simulink model "tb_power_plant"  (R2026b)
model workspace (MAT data in the model file):
  TB.do0_t = [0 0.01 10000000]
  TB.do0_v = [0 1 1]
  TB.do1_t = [0 0.03 0.08 10000000]
  TB.do1_v = [0 1 0 0]
  TB.k3_t = [0 10000000]
  TB.k3_v = [0 0]
  TB.duty_t = [0 10000000]
  TB.duty_v = [0 0]
  TB.noz_t = [0 10000000]
  TB.noz_v = [0 0]
  TB.lift_t = [0 10000000]
  TB.lift_v = [0 0]
  TB.estopF_t = [0 10000000]
  TB.estopF_v = [0 0]
  TB.estopR_t = [0 10000000]
  TB.estopR_v = [0 0]
  TB.wless_t = [0 10000000]
  TB.wless_v = [0 0]
  TB.bumpF_t = [0 10000000]
  TB.bumpF_v = [0 0]
  TB.bumpR_t = [0 10000000]
  TB.bumpR_v = [0 0]
  TB.reset_t = [0 10000000]
  TB.reset_v = [0 0]
  TB.keyoff_t = [0 10000000]
  TB.keyoff_v = [0 0]
  TB.ch2_t = [0 10000000]
  TB.ch2_v = [0 0]
  TB.bmsf_t = [0 10000000]
  TB.bmsf_v = [0 0]
  TB.hv_t = [0 1 10000000]
  TB.hv_v = [0 1 1]
  TB.chg_t = [0 10000000]
  TB.chg_v = [0 0]
  TB.rst_t = [0 10000000]
  TB.rst_v = [0 0]
  TB.sd_t = [0 10000000]
  TB.sd_v = [0 0]
  TB.alive_freeze_t = 1000000000
  TB.ien_t = [0 10000000]
  TB.ien_v = [0 0]
  TB.ispd_t = [0 10000000]
  TB.ispd_v = [0 0]
  TB.icmd_stop_t = 1000000000
  TB.P24_t = [0 10000000]
  TB.P24_v = [53 53]
  TB.P12_t = [0 10000000]
  TB.P12_v = [99 99]
  TB.P5_t = [0 10000000]
  TB.P5_v = [2.5 2.5]
  TB.P3_t = [0 10000000]
  TB.P3_v = [0.6 0.6]
  TB.T_amb = 298.15
  TB.G_solar = 0
  TB.dock_t = [0 10000000]
  TB.dock_v = [0 0]
  TB.C_drv = 0.0022
  TB.R_esr = 0.01
  TB.loadL_t = [0 10000000]
  TB.loadL_v = [0 0]
  TB.loadR_t = [0 10000000]
  TB.loadR_v = [0 0]
  TB.load_is_power = 0
  TB.V_gate = [30 35]
  TB.short_t = [0 10000000]
  TB.short_v = [0 0]
  TB.R_short = 0.005
  TB.J_impl = 0.05
  TB.k_aero = 1.19e-05
  TB.k_lin = 0
  TB.T_c = 0
  TB.k_lf = 0
  TB.lf_t = [0 10000000]
  TB.lf_v = [1 1]
  TB.p_line = 0
  TB.MaxNonlinIter = 3
  TB.MaxModeIter = 2
  TB.dec_fast = 1
  TB.dec_slow = 1
  TB.dec_bms = 1
  TB.dec_truth = 1
values from neighbouring files (symbols this model uses):
  P = local_temp(P, 318.15)    [pwr_case_def.m]    (also in pwr_case_run.m = C.pmod(P))
undefined symbols (not defined in the file or in its folder): bms_fault, estop_ch2_stuck, linePressure, shaftSpeed, shaftTorque, Ts, type, VC_IMPL
libraries: simulink x21, fl_lib x9, nesl_utility x8, ee_lib x4
settings Model: Creator=aomar  LastModifiedBy=aomar

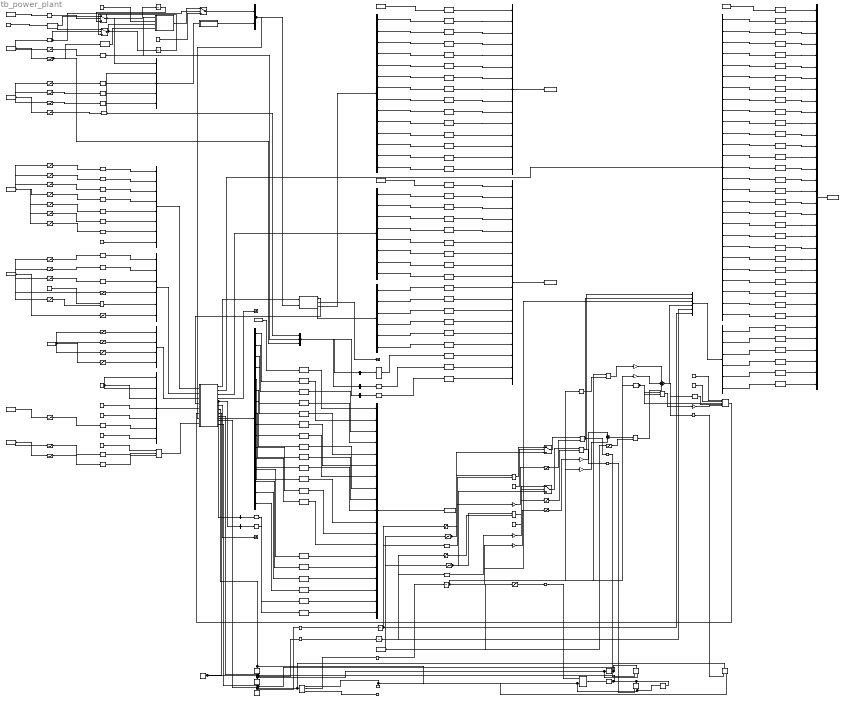
== system tb_power_plant ==
  Alive_cnt : simulink/Sources/Counter Free-Running  NumBits=8  tsamp=Ts.can_slow
  Alive_u8 : DataTypeConversion  OutDataTypeStr=uint8  SaturateOnIntegerOverflow=off  RndMeth=Floor
  Angle_term : fl_lib/Physical Signals/Sinks/PS Terminator
  BMS : ModelReference  ModelNameDialog=Shaddad_BMS  SimulationMode=Normal  ModelReferenceVersion=1.1
  BMS_REQ_Pack : Subsystem  ReferencedSubsystem=bmsreq_can_pack
  BmsReq_BC : BusCreator  Inputs=5  OutDataTypeStr=Bus: Bus_BmsReq  NonVirtualBus=on
      settings: InheritFromInputs=off
  Bms_alive_hold : UnitDelay  InitialCondition=uint8(0)  SampleTime=Ts.can_slow
  Bms_alive_run : simulink/Logic and Bit Operations/Compare To Constant  relop=<  const=TB.alive_freeze_t  OutDataTypeStr=boolean
  Bms_alive_sw : Switch  Criteria=u2 ~= 0  SaturateOnIntegerOverflow=off  InputSameDT=off
  C_drv_L : ee_lib/Passive/Capacitor  cap_option=ee.enum.passive.capacitor.capOption.const  c=TB.C_drv F  Cvec=[1e-05, 1e-06] F  Vvec=[0, 10] V  CV_table_symmetry=ee.enum.passive.capacitor.tableSymmetry.yes  f_vec=[1, 10] kHz  DFext_vec=[.8, 1.2]  enable_C_tol=ee.enum.toleranceApplication.none  averaging_period=0 s  C_tol=5  tol_distribution=ee.enum.toleranceDistribution.uniform  nSigma=4  r=TB.R_esr Ohm  g=0 1/Ohm  enable_operating_limits=ee.enum.enable.no  operating_limit_action=ee.enum.passive.reportOpLim.warn  max_working_voltage_range=[-25, 25] V  power_rating=1 W  maxTemperature=85 degC  thermalEnable=false  thermalMass=1 J/K  i_specify=off  i_priority=None  i=0 A  i_nominal_specify=off  i_nominal_value=1  i_nominal_unit=A  v_specify=off  v_priority=None  v=0 V  v_nominal_specify=off  v_nominal_value=1  v_nominal_unit=V  vc_specify=on  vc_priority=High  vc=0 V  vc_nominal_specify=off  vc_nominal_value=1  vc_nominal_unit=V  T_specify=off  T_priority=None  T=298.15 K  T_nominal_specify=off  T_nominal_value=1  T_nominal_unit=K
  C_drv_R : ee_lib/Passive/Capacitor  cap_option=ee.enum.passive.capacitor.capOption.const  c=TB.C_drv F  Cvec=[1e-05, 1e-06] F  Vvec=[0, 10] V  CV_table_symmetry=ee.enum.passive.capacitor.tableSymmetry.yes  f_vec=[1, 10] kHz  DFext_vec=[.8, 1.2]  enable_C_tol=ee.enum.toleranceApplication.none  averaging_period=0 s  C_tol=5  tol_distribution=ee.enum.toleranceDistribution.uniform  nSigma=4  r=TB.R_esr Ohm  g=0 1/Ohm  enable_operating_limits=ee.enum.enable.no  operating_limit_action=ee.enum.passive.reportOpLim.warn  max_working_voltage_range=[-25, 25] V  power_rating=1 W  maxTemperature=85 degC  thermalEnable=false  thermalMass=1 J/K  i_specify=off  i_priority=None  i=0 A  i_nominal_specify=off  i_nominal_value=1  i_nominal_unit=A  v_specify=off  v_priority=None  v=0 V  v_nominal_specify=off  v_nominal_value=1  v_nominal_unit=V  vc_specify=on  vc_priority=High  vc=0 V  vc_nominal_specify=off  vc_nominal_value=1  vc_nominal_unit=V  T_specify=off  T_priority=None  T=298.15 K  T_nominal_specify=off  T_nominal_value=1  T_nominal_unit=K
  CanSlow_BC : BusCreator  Inputs=2  OutDataTypeStr=Bus: Bus_Can1_McuSlow  NonVirtualBus=on
      settings: InheritFromInputs=off
  Clock_100ms : DigitalClock  SampleTime=Ts.env
  Clock_100ms_log : DigitalClock  SampleTime=Ts.hk
  Clock_100ms_log_bms : DigitalClock  SampleTime=Ts.hk
  Clock_10ms : DigitalClock  SampleTime=Ts.ctrl
  Clock_10ms_lv : DigitalClock  SampleTime=Ts.ctrl
  Clock_50ms : DigitalClock  SampleTime=Ts.can_slow
  Clock_50ms_alive : DigitalClock  SampleTime=Ts.can_slow
  Clock_50ms_impl : DigitalClock  SampleTime=Ts.can_slow
  Clock_base : DigitalClock  SampleTime=Ts.base
  Clock_base_flt : DigitalClock  SampleTime=Ts.base
  Clock_base_hmi : DigitalClock  SampleTime=Ts.base
  Clock_base_hw : DigitalClock  SampleTime=Ts.base
  Clock_base_stub : DigitalClock  SampleTime=Ts.base
  Cmd_sel : BusSelector  OutputSignals=K1_Cmd,K2_Cmd,K4_Cmd,Charger_Enable,Charger_I_Req_A,Fan_Cmd
  Dist : Constant  Value=0  SampleTime=Ts.env
  Env_BC : BusCreator  Inputs=7  OutDataTypeStr=Bus: Bus_EnvState  NonVirtualBus=on
      settings: InheritFromInputs=off
  Flt_BA : BusAssignment  AssignedSignals=estop_ch2_stuck,bms_fault
  Flt_ic : Constant  Value=P.ic.Bus_FaultInject  OutDataTypeStr=Bus: Bus_FaultInject  SampleTime=Ts.base
  G_solar : Constant  Value=TB.G_solar  SampleTime=Ts.env
  Gate_L : Saturate  UpperLimit=1  LowerLimit=0
  Gate_L_k : Gain  Gain=1/(TB.V_gate(2) - TB.V_gate(1))
  Gate_L_off : Bias  Bias=-TB.V_gate(1)  SaturateOnIntegerOverflow=off
  Gate_R : Saturate  UpperLimit=1  LowerLimit=0
  Gate_R_k : Gain  Gain=1/(TB.V_gate(2) - TB.V_gate(1))
  Gate_R_off : Bias  Bias=-TB.V_gate(1)  SaturateOnIntegerOverflow=off
  Hmi_BC : BusCreator  Inputs=8  OutDataTypeStr=Bus: Bus_HmiInputs  NonVirtualBus=on
      settings: InheritFromInputs=off
  Hv_RT : RateTransition  OutPortSampleTime=Ts.ctrl
  Hv_log_sel : BusSelector  OutputSignals=HV_Enable_Req
  Hw_BC : BusCreator  Inputs=6  OutDataTypeStr=Bus: Bus_PowerHwCmd  NonVirtualBus=on
      settings: InheritFromInputs=off
  IMPL_CMD_Pack : Subsystem  ReferencedSubsystem=implcmd_can_pack
  I_drv_L : fl_lib/Electrical/Electrical Sources/Controlled Current Source
  I_drv_L_PS : nesl_utility/Simulink-PS Converter  PhysicalDomain=network_engine_domain  SubClassName=ps_input  LeftPortType=input  RightPortType=output  PseudoPeriodic=off  Frequencies=[]  NoiseDistribution=none  NoiseParameters=[]  Unit=A  AffineConversion=off  FilteringAndDerivatives=zero  SimscapeFilterOrder=1  InputFilterTimeConstant=0.001  UdotUserProvided=0
  I_drv_R : fl_lib/Electrical/Electrical Sources/Controlled Current Source
  I_drv_R_PS : nesl_utility/Simulink-PS Converter  PhysicalDomain=network_engine_domain  SubClassName=ps_input  LeftPortType=input  RightPortType=output  PseudoPeriodic=off  Frequencies=[]  NoiseDistribution=none  NoiseParameters=[]  Unit=A  AffineConversion=off  FilteringAndDerivatives=zero  SimscapeFilterOrder=1  InputFilterTimeConstant=0.001  UdotUserProvided=0
  I_from_P_L : Product  Inputs=*/
  I_from_P_R : Product  Inputs=*/
  I_load_L : Product
  I_load_R : Product
  Icmd_alive_hold : UnitDelay  InitialCondition=uint8(0)  SampleTime=Ts.can_slow
  Icmd_alive_sw : Switch  Criteria=u2 ~= 0  SaturateOnIntegerOverflow=off  InputSameDT=off
  Icmd_none : Constant  Value=P.ic.Bus_CanFrame8  OutDataTypeStr=Bus: Bus_CanFrame8  SampleTime=Ts.can_slow
  Icmd_rst : Constant  Value=false  OutDataTypeStr=boolean  SampleTime=Ts.can_slow
  Icmd_run : simulink/Logic and Bit Operations/Compare To Constant  relop=<  const=TB.icmd_stop_t  OutDataTypeStr=boolean
  Icmd_valid : Switch  Criteria=u2 ~= 0  SaturateOnIntegerOverflow=off  InputSameDT=off
  Ien_RT : RateTransition  OutPortSampleTime=Ts.ctrl
  Ien_log_sel : BusSelector  OutputSignals=impl_enable
  Impl_sel : BusSelector  OutputSignals=Impl_Running,Impl_Fault,Impl_Ready,Impl_Speed_radps,Impl_Torque_Nm,Impl_Power_W,Impl_Current_A,Fault_Code
  Impl_type : Constant  Value=uint8(VC_IMPL)  OutDataTypeStr=uint8  SampleTime=Ts.ctrl
  Is_power_L : Constant  Value=TB.load_is_power  SampleTime=Ts.base
  Is_power_R : Constant  Value=TB.load_is_power  SampleTime=Ts.base
  Ispd_RT : RateTransition  OutPortSampleTime=Ts.ctrl
  Ispd_log_sel : BusSelector  OutputSignals=impl_speed_rpm
  Ispd_s : DataTypeConversion  OutDataTypeStr=single  SaturateOnIntegerOverflow=off  RndMeth=Floor
  J_impl : fl_lib/Mechanical/Rotational Elements/Inertia  inertia=TB.J_impl kg*m^2  num_ports=foundation.enum.numPorts2.one  w_specify=off  w_priority=High  w=0 rad/s  w_nominal_specify=off  w_nominal_value=1  w_nominal_unit=rad/s  t_specify=off  t_priority=None  t=0 N*m  t_nominal_specify=off  t_nominal_value=1  t_nominal_unit=N*m
  K_aero : Gain  Gain=TB.k_aero
  K_lf : Gain  Gain=TB.k_lf
  K_lin : Gain  Gain=TB.k_lin
  LF : Lookup_n-D  NumberOfTableDimensions=1  BreakpointsForDimension1=TB.lf_t  Table=TB.lf_v  InterpMethod=Flat  ExtrapMethod=Clip  InternalRulePriority=Speed  RndMeth=Simplest
  Load_L : Lookup_n-D  NumberOfTableDimensions=1  BreakpointsForDimension1=TB.loadL_t  Table=TB.loadL_v  InterpMethod=Flat  ExtrapMethod=Clip  InternalRulePriority=Speed  RndMeth=Simplest
  Load_R : Lookup_n-D  NumberOfTableDimensions=1  BreakpointsForDimension1=TB.loadR_t  Table=TB.loadR_v  InterpMethod=Flat  ExtrapMethod=Clip  InternalRulePriority=Speed  RndMeth=Simplest
  Load_mode_L : Switch  Criteria=u2 ~= 0  SaturateOnIntegerOverflow=off  InputSameDT=off
  Load_mode_R : Switch  Criteria=u2 ~= 0  SaturateOnIntegerOverflow=off  InputSameDT=off
  Lv_BC : BusCreator  Inputs=4  OutDataTypeStr=Bus: Bus_LV_LoadDemand  NonVirtualBus=on
      settings: InheritFromInputs=off
  Mcu_log_BC : BusCreator  Inputs=3
  Mech_BA : BusAssignment  AssignedSignals=type,shaftSpeed,shaftTorque,linePressure
  Mech_ic : Constant  Value=P.ic.Bus_ImplMechState  OutDataTypeStr=Bus: Bus_ImplMechState  SampleTime=Ts.ctrl
  Noz_idx : Constant  Value=(1:8)'  SampleTime=Ts.base
  Noz_on : RelationalOperator  Operator=<=  OutDataTypeStr=boolean  RndMeth=Simplest  InputSameDT=off
  P_line : Gain  Gain=TB.p_line*P.structure.impl.sprayer.p_set/P.power.impl.sprayer.w_nom^2
  Power_Plant : Subsystem  ReferencedSubsystem=Power_Plant
  R_short : ee_lib/Passive/Resistor  R=TB.R_short Ohm  enable_R_tol=ee.enum.toleranceApplication.none  R_tol=5  tol_distribution=ee.enum.toleranceDistribution.uniform  nSigma=4  enable_operating_limits=ee.enum.enable.no  operating_limit_action=ee.enum.passive.reportOpLim.warn  power_rating=1 W  max_working_voltage=100 V  noise_mode=ee.enum.sources.noise.Disabled  Tdevice=25 degC  sample_time=1e-3 s  repeatability=ee.enum.ic.repeatability.notRepeatable  user_seed=0  auto_seed=216421012  power_derating_T1=70 degC  power_derating_T2=155 degC  operating_temperature_range_vec=[-50, 150] degC  alpha=3.93e-3 1/K  Tmeas=25 degC  thermal_mass=100 J/K  temperature_specify=off  temperature_priority=High  temperature=298.15 K  temperature_nominal_specify=off  temperature_nominal_value=1  temperature_nominal_unit=K
  Ref_impl : fl_lib/Mechanical/Rotational Elements/Mechanical Rotational Reference
  SOC_true_min : MinMax
  SOC_true_sel : BusSelector  OutputSignals=SOC_true
  S_short : ee_lib/Switches & Breakers/SPST Switch  R_closed=1e-6 Ohm  G_open=1e-8 S  Threshold=0.5 V  Width=0 V  model_dynamics=0  t_on=1e-3 s  t_off=1e-3 s  initial_vT=0 V
  Short : Lookup_n-D  NumberOfTableDimensions=1  BreakpointsForDimension1=TB.short_t  Table=TB.short_v  InterpMethod=Flat  ExtrapMethod=Clip  InternalRulePriority=Speed  RndMeth=Simplest
  Short_PS : nesl_utility/Simulink-PS Converter  PhysicalDomain=network_engine_domain  SubClassName=ps_input  LeftPortType=input  RightPortType=output  PseudoPeriodic=off  Frequencies=[]  NoiseDistribution=none  NoiseParameters=[]  Unit=V  AffineConversion=off  FilteringAndDerivatives=zero  SimscapeFilterOrder=1  InputFilterTimeConstant=0.001  UdotUserProvided=0
  Soil : Constant  Value=uint8(1)  OutDataTypeStr=uint8  SampleTime=Ts.env
  Solver : nesl_utility/Solver Configuration  PhysicalDomain=network_engine_domain  SubClassName=solver  LeftPortType=input  RightPortType=generic  Tones=[]  Harmonics=[]  SimulateNoise=off  Profile=off  UseLocalSampling=off  EnableSwitchedLinearOptims=on  FrequencyDomain=off  UseCCode=off  RelTol=0.001  AbsTol=0.001  MinStep=1e-09  ToWorkspace=off  RevertToSquareIcSolve=off  NumHomotopyIterations=100  PhasorMode=off  PhasorModeNumHarmonics=1  ConsistencySolver=NEWTON_XTOL_AFTER_FTOL  CanonicalOrdering=CANONICAL  OptimizeIntermediates=OPTIMIZED  MulticoreSolverChoice=BACKWARD_EULER  IndexReductionMethod=DerivativeReplacement  DoDC=off  ResidualTolerance=1e-09  ConsistencyTolSource=GLOBAL  ConsistencyAbsTol=0.001  ConsistencyRelTol=0.001  ConsistencyTolFactor=0.001  UseLocalSolver=on  LocalSolverChoice=NE_BACKWARD_EULER_ADVANCER  ResolveIndetEquations=on  FunctionEvalNumThread=1  LocalSolverSampleTime=P.sim.ssc.Ts  DoFixedCost=on  MaxNonlinIter=TB.MaxNonlinIter  MaxModeIter=TB.MaxModeIter  ComputeImpulses=off  ImpulseIterations=2  LinearAlgebra=auto  LinearAlgebraNumThread=0  EquationFormulation=NE_TIME_EF  DelaysMemoryBudget=1024  AutomaticFiltering=on  FilteringTimeConstant=0.001  PartitionStorageMethod=AS_NEEDED  PartitionMemoryBudget=1024  PartitionMethod=BALANCED  MultibodyUseLocalSolver=off  MultibodyLocalSolverChoice=ODE1  MultibodyLocalSolverSampleTime=0.001
  Status_sel : BusSelector  OutputSignals=V_pack_V,I_pack_A,V_bus_V,V_24V_V,I_24V_A,V_24IMP_V,V_12V_V,I_12V_A,V_5V_V,V_3V3_V,Rail_24V_OK,Rail_12V_OK,Rail_5V_OK,Rail_3V3_OK,K1_Closed,K2_Closed,K3_Closed,K4_Closed,Safety_OK,Safety_HV_OK,EStop_Any,EStop_Ch1_OK,EStop_Ch2_OK,Safety_Latched_Off,Dock_Present,Key_On,Fuse_Blown
  Stub_log_BC : BusCreator  Inputs=6
  Stub_log_sel : BusSelector  OutputSignals=I_load_L,I_load_R,w_impl_d,T_load,V_drv_L_d,V_drv_R_d
  T_amb : Constant  Value=TB.T_amb  SampleTime=Ts.env
  T_c : Gain  Gain=TB.T_c
  T_lf : Product
  T_lf_sum : Sum
  T_load : Sum  Inputs=---
  T_load_PS : nesl_utility/Simulink-PS Converter  PhysicalDomain=network_engine_domain  SubClassName=ps_input  LeftPortType=input  RightPortType=output  PseudoPeriodic=off  Frequencies=[]  NoiseDistribution=none  NoiseParameters=[]  Unit=N*m  AffineConversion=off  FilteringAndDerivatives=zero  SimscapeFilterOrder=1  InputFilterTimeConstant=0.001  UdotUserProvided=0
  T_load_RT : RateTransition  OutPortSampleTime=Ts.ctrl
  T_load_src : fl_lib/Mechanical/Mechanical Sources/Ideal Torque Source
  Tel_sel : BusSelector  OutputSignals=Contactor_State,HV_Ready,Fault_Level,Fault_Word,Warning_Word,SOC_pack,Charging_Active,Charge_Complete,I_chg_lim_A,I_dis_lim_A,T_cell_max_K,Fan_Cmd,K1_Closed,Runtime_Remaining_s
  Truth_sel : BusSelector  OutputSignals=SOC_pack_true,T_cell_max_K,T_cell_min_K,V_term_V,I_pack_A,E_out_Wh,E_in_Wh,E_chg_bus_Wh,E_trac_dc_Wh,E_impl_dc_Wh,E_lv_Wh,E_dcdc_loss_Wh,E_pdu_loss_Wh,E_loss_batt_Wh,I_pack_peak_A,P_grid_W
  V_L_min : Saturate  UpperLimit=inf  LowerLimit=30
  V_R_min : Saturate  UpperLimit=inf  LowerLimit=30
  V_cell_true_max : MinMax  Function=max
  V_cell_true_sel : BusSelector  OutputSignals=V_cell_true
  V_drv_L : nesl_utility/PS-Simulink Converter  PhysicalDomain=network_engine_domain  SubClassName=ps_output  LeftPortType=input  RightPortType=output  PseudoPeriodic=off  Frequencies=[]  VectorFormat=inherit  Unit=V  AffineConversion=off
  V_drv_L_d : UnitDelay  SampleTime=Ts.base
  V_drv_L_sens : fl_lib/Electrical/Electrical Sensors/Voltage Sensor
  V_drv_R : nesl_utility/PS-Simulink Converter  PhysicalDomain=network_engine_domain  SubClassName=ps_output  LeftPortType=input  RightPortType=output  PseudoPeriodic=off  Frequencies=[]  VectorFormat=inherit  Unit=V  AffineConversion=off
  V_drv_R_d : UnitDelay  SampleTime=Ts.base
  V_drv_R_sens : fl_lib/Electrical/Electrical Sensors/Voltage Sensor
  W_10 : Gain  Gain=0.1
  W_abs : Abs  SaturateOnIntegerOverflow=off
  W_impl : nesl_utility/PS-Simulink Converter  PhysicalDomain=network_engine_domain  SubClassName=ps_output  LeftPortType=input  RightPortType=output  PseudoPeriodic=off  Frequencies=[]  VectorFormat=inherit  Unit=rad/s  AffineConversion=off
  W_impl_RT : RateTransition  OutPortSampleTime=Ts.ctrl
  W_impl_d : UnitDelay  SampleTime=Ts.base
  W_impl_sens : fl_lib/Mechanical/Mechanical Sensors/Ideal Rotational Motion Sensor  reference=foundation.enum.MeasurementReference.difference  acceleration_port=false  velocity_port=true  position_port=true  wrap_angle=false  offset=0 rad
  W_sat : Saturate  UpperLimit=1  LowerLimit=-1
  W_sq : Product
  W_sq_p : Product
  can_tx_bms_term : Terminator
  env_dock : simulink/Logic and Bit Operations/Compare To Zero  relop=~=  OutDataTypeStr=boolean
  env_dock_tab : Lookup_n-D  NumberOfTableDimensions=1  BreakpointsForDimension1=TB.dock_t  Table=TB.dock_v  InterpMethod=Flat  ExtrapMethod=Clip  InternalRulePriority=Speed  RndMeth=Simplest
  flt_bms : simulink/Logic and Bit Operations/Compare To Zero  relop=~=  OutDataTypeStr=boolean
  flt_bms_tab : Lookup_n-D  NumberOfTableDimensions=1  BreakpointsForDimension1=TB.bmsf_t  Table=TB.bmsf_v  InterpMethod=Flat  ExtrapMethod=Clip  InternalRulePriority=Speed  RndMeth=Simplest
  flt_ch2 : simulink/Logic and Bit Operations/Compare To Zero  relop=~=  OutDataTypeStr=boolean
  flt_ch2_tab : Lookup_n-D  NumberOfTableDimensions=1  BreakpointsForDimension1=TB.ch2_t  Table=TB.ch2_v  InterpMethod=Flat  ExtrapMethod=Clip  InternalRulePriority=Speed  RndMeth=Simplest
  hmi_bumpF : simulink/Logic and Bit Operations/Compare To Zero  relop=~=  OutDataTypeStr=boolean
  hmi_bumpF_tab : Lookup_n-D  NumberOfTableDimensions=1  BreakpointsForDimension1=TB.bumpF_t  Table=TB.bumpF_v  InterpMethod=Flat  ExtrapMethod=Clip  InternalRulePriority=Speed  RndMeth=Simplest
  hmi_bumpR : simulink/Logic and Bit Operations/Compare To Zero  relop=~=  OutDataTypeStr=boolean
  hmi_bumpR_tab : Lookup_n-D  NumberOfTableDimensions=1  BreakpointsForDimension1=TB.bumpR_t  Table=TB.bumpR_v  InterpMethod=Flat  ExtrapMethod=Clip  InternalRulePriority=Speed  RndMeth=Simplest
  hmi_estopF : simulink/Logic and Bit Operations/Compare To Zero  relop=~=  OutDataTypeStr=boolean
  hmi_estopF_tab : Lookup_n-D  NumberOfTableDimensions=1  BreakpointsForDimension1=TB.estopF_t  Table=TB.estopF_v  InterpMethod=Flat  ExtrapMethod=Clip  InternalRulePriority=Speed  RndMeth=Simplest
  hmi_estopR : simulink/Logic and Bit Operations/Compare To Zero  relop=~=  OutDataTypeStr=boolean
  hmi_estopR_tab : Lookup_n-D  NumberOfTableDimensions=1  BreakpointsForDimension1=TB.estopR_t  Table=TB.estopR_v  InterpMethod=Flat  ExtrapMethod=Clip  InternalRulePriority=Speed  RndMeth=Simplest
  hmi_keyoff : simulink/Logic and Bit Operations/Compare To Zero  relop=~=  OutDataTypeStr=boolean
  hmi_keyoff_tab : Lookup_n-D  NumberOfTableDimensions=1  BreakpointsForDimension1=TB.keyoff_t  Table=TB.keyoff_v  InterpMethod=Flat  ExtrapMethod=Clip  InternalRulePriority=Speed  RndMeth=Simplest
  hmi_lid : Constant  Value=false  OutDataTypeStr=boolean  SampleTime=Ts.base
  hmi_reset : simulink/Logic and Bit Operations/Compare To Zero  relop=~=  OutDataTypeStr=boolean
  hmi_reset_tab : Lookup_n-D  NumberOfTableDimensions=1  BreakpointsForDimension1=TB.reset_t  Table=TB.reset_v  InterpMethod=Flat  ExtrapMethod=Clip  InternalRulePriority=Speed  RndMeth=Simplest
  hmi_wless : simulink/Logic and Bit Operations/Compare To Zero  relop=~=  OutDataTypeStr=boolean
  hmi_wless_tab : Lookup_n-D  NumberOfTableDimensions=1  BreakpointsForDimension1=TB.wless_t  Table=TB.wless_v  InterpMethod=Flat  ExtrapMethod=Clip  InternalRulePriority=Speed  RndMeth=Simplest
  hw_do0 : simulink/Logic and Bit Operations/Compare To Zero  relop=~=  OutDataTypeStr=boolean
  hw_do0_tab : Lookup_n-D  NumberOfTableDimensions=1  BreakpointsForDimension1=TB.do0_t  Table=TB.do0_v  InterpMethod=Flat  ExtrapMethod=Clip  InternalRulePriority=Speed  RndMeth=Simplest
  hw_do1 : simulink/Logic and Bit Operations/Compare To Zero  relop=~=  OutDataTypeStr=boolean
  hw_do1_tab : Lookup_n-D  NumberOfTableDimensions=1  BreakpointsForDimension1=TB.do1_t  Table=TB.do1_v  InterpMethod=Flat  ExtrapMethod=Clip  InternalRulePriority=Speed  RndMeth=Simplest
  hw_duty : Lookup_n-D  NumberOfTableDimensions=1  BreakpointsForDimension1=TB.duty_t  Table=TB.duty_v  InterpMethod=Flat  ExtrapMethod=Clip  InternalRulePriority=Speed  RndMeth=Simplest
  hw_k3 : simulink/Logic and Bit Operations/Compare To Zero  relop=~=  OutDataTypeStr=boolean
  hw_k3_tab : Lookup_n-D  NumberOfTableDimensions=1  BreakpointsForDimension1=TB.k3_t  Table=TB.k3_v  InterpMethod=Flat  ExtrapMethod=Clip  InternalRulePriority=Speed  RndMeth=Simplest
  hw_lift : Lookup_n-D  NumberOfTableDimensions=1  BreakpointsForDimension1=TB.lift_t  Table=TB.lift_v  InterpMethod=Flat  ExtrapMethod=Clip  InternalRulePriority=Speed  RndMeth=Simplest
  hw_noz : Lookup_n-D  NumberOfTableDimensions=1  BreakpointsForDimension1=TB.noz_t  Table=TB.noz_v  InterpMethod=Flat  ExtrapMethod=Clip  InternalRulePriority=Speed  RndMeth=Simplest
  impl_can_term : Terminator
  lb_dbl{1..15} (15 alike) : DataTypeConversion  OutDataTypeStr=double  SaturateOnIntegerOverflow=off  RndMeth=Floor
  lf_dbl{1..34} (34 alike) : DataTypeConversion  OutDataTypeStr=double  SaturateOnIntegerOverflow=off  RndMeth=Floor
  log_bms : ToWorkspace  VariableName=log_bms  SampleTime=-1
      settings: Decimation=TB.dec_bms
  log_bms_mux : Mux  Inputs=15
  log_fast : ToWorkspace  VariableName=log_fast  SampleTime=-1
      settings: Decimation=TB.dec_fast
  log_fast_mux : Mux  Inputs=34
  log_slow : ToWorkspace  VariableName=log_slow  SampleTime=-1
      settings: Decimation=TB.dec_slow
  log_slow_mux : Mux  Inputs=18
  log_truth : ToWorkspace  VariableName=log_truth  SampleTime=-1
      settings: Decimation=TB.dec_truth
  log_truth_mux : Mux  Inputs=19
  ls_dbl{1..18} (18 alike) : DataTypeConversion  OutDataTypeStr=double  SaturateOnIntegerOverflow=off  RndMeth=Floor
  lt_dbl{1..19} (19 alike) : DataTypeConversion  OutDataTypeStr=double  SaturateOnIntegerOverflow=off  RndMeth=Floor
  lv_P12 : Lookup_n-D  NumberOfTableDimensions=1  BreakpointsForDimension1=TB.P12_t  Table=TB.P12_v  InterpMethod=Flat  ExtrapMethod=Clip  InternalRulePriority=Speed  RndMeth=Simplest
  lv_P24 : Lookup_n-D  NumberOfTableDimensions=1  BreakpointsForDimension1=TB.P24_t  Table=TB.P24_v  InterpMethod=Flat  ExtrapMethod=Clip  InternalRulePriority=Speed  RndMeth=Simplest
  lv_P3 : Lookup_n-D  NumberOfTableDimensions=1  BreakpointsForDimension1=TB.P3_t  Table=TB.P3_v  InterpMethod=Flat  ExtrapMethod=Clip  InternalRulePriority=Speed  RndMeth=Simplest
  lv_P5 : Lookup_n-D  NumberOfTableDimensions=1  BreakpointsForDimension1=TB.P5_t  Table=TB.P5_v  InterpMethod=Flat  ExtrapMethod=Clip  InternalRulePriority=Speed  RndMeth=Simplest
  mcu_chg : simulink/Logic and Bit Operations/Compare To Zero  relop=~=  OutDataTypeStr=boolean
  mcu_chg_tab : Lookup_n-D  NumberOfTableDimensions=1  BreakpointsForDimension1=TB.chg_t  Table=TB.chg_v  InterpMethod=Flat  ExtrapMethod=Clip  InternalRulePriority=Speed  RndMeth=Simplest
  mcu_hv : simulink/Logic and Bit Operations/Compare To Zero  relop=~=  OutDataTypeStr=boolean
  mcu_hv_tab : Lookup_n-D  NumberOfTableDimensions=1  BreakpointsForDimension1=TB.hv_t  Table=TB.hv_v  InterpMethod=Flat  ExtrapMethod=Clip  InternalRulePriority=Speed  RndMeth=Simplest
  mcu_ien : simulink/Logic and Bit Operations/Compare To Zero  relop=~=  OutDataTypeStr=boolean
  mcu_ien_tab : Lookup_n-D  NumberOfTableDimensions=1  BreakpointsForDimension1=TB.ien_t  Table=TB.ien_v  InterpMethod=Flat  ExtrapMethod=Clip  InternalRulePriority=Speed  RndMeth=Simplest
  mcu_ispd : Lookup_n-D  NumberOfTableDimensions=1  BreakpointsForDimension1=TB.ispd_t  Table=TB.ispd_v  InterpMethod=Flat  ExtrapMethod=Clip  InternalRulePriority=Speed  RndMeth=Simplest
  mcu_rst : simulink/Logic and Bit Operations/Compare To Zero  relop=~=  OutDataTypeStr=boolean
  mcu_rst_tab : Lookup_n-D  NumberOfTableDimensions=1  BreakpointsForDimension1=TB.rst_t  Table=TB.rst_v  InterpMethod=Flat  ExtrapMethod=Clip  InternalRulePriority=Speed  RndMeth=Simplest
  mcu_sd : simulink/Logic and Bit Operations/Compare To Zero  relop=~=  OutDataTypeStr=boolean
  mcu_sd_tab : Lookup_n-D  NumberOfTableDimensions=1  BreakpointsForDimension1=TB.sd_t  Table=TB.sd_v  InterpMethod=Flat  ExtrapMethod=Clip  InternalRulePriority=Speed  RndMeth=Simplest
  safety_term : Terminator
  wires:
  Alive_cnt/1 -> Alive_u8/1  "alive_count"
  Clock_50ms_alive/1 -> Bms_alive_run/1  "t_50ms_alive"
  Clock_50ms_impl/1 -> mcu_ispd/1, Icmd_run/1, mcu_ien_tab/1  "t_50ms_impl"
  Clock_50ms/1 -> mcu_hv_tab/1, mcu_chg_tab/1, mcu_sd_tab/1, mcu_rst_tab/1  "t_50ms"
  Clock_base_hmi/1 -> hmi_keyoff_tab/1, hmi_reset_tab/1, hmi_estopF_tab/1, hmi_bumpR_tab/1, hmi_estopR_tab/1, hmi_bumpF_tab/1, hmi_wless_tab/1  "t_base_hmi"
  Clock_base_hw/1 -> hw_lift/1, hw_noz/1, hw_duty/1, hw_do0_tab/1, hw_do1_tab/1, hw_k3_tab/1  "t_base_hw"
  Clock_100ms/1 -> env_dock_tab/1  "t_100ms"
  Clock_base_flt/1 -> flt_bms_tab/1, flt_ch2_tab/1  "t_base_flt"
  Bms_alive_run/1 -> Bms_alive_sw/2  "bms_alive_run"
  Icmd_run/1 -> Icmd_valid/2, Icmd_alive_sw/2  "impl_cmd_run"
  Noz_idx/1 -> Noz_on/1  "nozzle_index"
  mcu_ien_tab/1 -> mcu_ien/1  "mcu_ien_tab"
  mcu_ispd/1 -> Mcu_log_BC/3, Ispd_s/1  "impl_speed_rpm"
  mcu_chg_tab/1 -> mcu_chg/1  "mcu_chg_tab"
  mcu_rst_tab/1 -> mcu_rst/1  "mcu_rst_tab"
  mcu_sd_tab/1 -> mcu_sd/1  "mcu_sd_tab"
  mcu_hv_tab/1 -> mcu_hv/1  "mcu_hv_tab"
  hmi_estopF_tab/1 -> hmi_estopF/1  "hmi_estopF_tab"
  hmi_estopR_tab/1 -> hmi_estopR/1  "hmi_estopR_tab"
  hmi_wless_tab/1 -> hmi_wless/1  "hmi_wless_tab"
  hmi_bumpF_tab/1 -> hmi_bumpF/1  "hmi_bumpF_tab"
  hmi_bumpR_tab/1 -> hmi_bumpR/1  "hmi_bumpR_tab"
  hmi_reset_tab/1 -> hmi_reset/1  "hmi_reset_tab"
  hmi_keyoff_tab/1 -> hmi_keyoff/1  "hmi_keyoff_tab"
  hw_do0_tab/1 -> hw_do0/1  "hw_do0_tab"
  hw_do1_tab/1 -> hw_do1/1  "hw_do1_tab"
  hw_k3_tab/1 -> hw_k3/1  "hw_k3_tab"
  hw_noz/1 -> Noz_on/2  "nozzles_on_count"
  env_dock_tab/1 -> env_dock/1  "env_dock_tab"
  flt_ch2_tab/1 -> flt_ch2/1  "flt_ch2_tab"
  flt_bms_tab/1 -> flt_bms/1  "flt_bms_tab"
  Clock_10ms_lv/1 -> lv_P3/1, lv_P24/1, lv_P5/1, lv_P12/1  "t_10ms_lv"
  Alive_u8/1 -> Bms_alive_sw/1, Icmd_alive_sw/1  "alive_u8"
  Icmd_rst/1 -> IMPL_CMD_Pack/2  "impl_fault_reset"
  hmi_lid/1 -> Hmi_BC/8  "lid_open"
  Noz_on/1 -> Hw_BC/5  "Spray_Nozzle_Cmd"
  T_amb/1 -> Env_BC/3, Env_BC/1, Env_BC/2  "T_ground"
  G_solar/1 -> Env_BC/4  "G_solar"
  Soil/1 -> Env_BC/5  "soil_id"
  Dist/1 -> Env_BC/7  "dist_dock"
  Flt_ic/1 -> Flt_BA/1  "flt_ic"
  mcu_ien/1 -> Mcu_log_BC/2, IMPL_CMD_Pack/1  "impl_enable"
  mcu_chg/1 -> BmsReq_BC/3  "Charge_Enable_Req"
  mcu_rst/1 -> BmsReq_BC/4  "Fault_Reset_Req"
  mcu_sd/1 -> BmsReq_BC/5  "Shutdown_Req"
  hmi_estopF/1 -> Hmi_BC/1  "estop_front_pressed"
  hmi_estopR/1 -> Hmi_BC/2  "estop_rear_pressed"
  hmi_wless/1 -> Hmi_BC/3  "wireless_estop_tripped"
  hmi_bumpF/1 -> Hmi_BC/4  "bumper_front"
  hmi_bumpR/1 -> Hmi_BC/5  "bumper_rear"
  hmi_reset/1 -> Hmi_BC/6  "reset_btn"
  hmi_keyoff/1 -> Hmi_BC/7  "key_off"
  hw_do0/1 -> Hw_BC/1  "MCU_Safety_OK"
  hw_do1/1 -> Hw_BC/2  "Safety_Reset_Req"
  hw_k3/1 -> Hw_BC/3  "ImpPwr24_Enable"
  hw_duty/1 -> Hw_BC/4  "Spray_Pump_Duty"
  hw_lift/1 -> Hw_BC/6  "Lift_Duty"
  lv_P24/1 -> Lv_BC/1  "P_24V_W"
  lv_P12/1 -> Lv_BC/2  "P_12V_W"
  lv_P5/1 -> Lv_BC/3  "P_5V_W"
  lv_P3/1 -> Lv_BC/4  "P_3V3_W"
  env_dock/1 -> Env_BC/6  "dock_contact"
  flt_ch2/1 -> Flt_BA/2  "estop_ch2_stuck"
  flt_bms/1 -> Flt_BA/3  "bms_fault"
  Bms_alive_sw/1 -> BmsReq_BC/1, Bms_alive_hold/1  "AliveCounter"
  mcu_hv/1 -> Mcu_log_BC/1, BmsReq_BC/2  "HV_Enable_Req"
  Icmd_alive_sw/1 -> Icmd_alive_hold/1, IMPL_CMD_Pack/3  "impl_alive"
  Ispd_s/1 -> IMPL_CMD_Pack/4  "impl_speed_rpm_s"
  BmsReq_BC/1 -> BMS_REQ_Pack/1  "bms_req"
  Hmi_BC/1 -> Power_Plant/1  "hmi"
  Hw_BC/1 -> Power_Plant/2  "hw_cmd"
  Lv_BC/1 -> Power_Plant/3  "lv_demand"
  Env_BC/1 -> Power_Plant/5  "env"
  Icmd_none/1 -> Icmd_valid/3  "impl_cmd_none"
  Bms_alive_hold/1 -> Bms_alive_sw/3  "bms_alive_held"
  Icmd_alive_hold/1 -> Icmd_alive_sw/3  "impl_alive_held"
  Flt_BA/1 -> Power_Plant/8  "flt"
  IMPL_CMD_Pack/1 -> Icmd_valid/1  "impl_cmd_frame"
  Icmd_valid/1 -> CanSlow_BC/1  "impl_cmd"
  BMS_REQ_Pack/1 -> CanSlow_BC/2  "bms_req"
  Power_Plant/1 -> BMS/1  "bms_meas"
  Power_Plant/2 -> Status_sel/1  "power_status"
  Power_Plant/3 -> Impl_sel/1  "impl_elec"
  Power_Plant/4 -> impl_can_term/1  "can_tx_impl"
  Power_Plant/5 -> V_cell_true_sel/1, SOC_true_sel/1, Truth_sel/1  "power_truth"
  Power_Plant/6 -> safety_term/1  "safety_ok"
  SOC_true_sel/1 -> SOC_true_min/1  "<SOC_true>"
  V_cell_true_sel/1 -> V_cell_true_max/1  "<V_cell_true>"
  CanSlow_BC/1 -> Power_Plant/7, BMS/2  "can_rx"
  Truth_sel/1 -> lt_dbl2/1  "<SOC_pack_true>"
  Truth_sel/2 -> lt_dbl3/1  "<T_cell_max_K>"
  Truth_sel/3 -> lt_dbl4/1  "<T_cell_min_K>"
  Truth_sel/4 -> lt_dbl5/1  "<V_term_V>"
  Truth_sel/5 -> lt_dbl6/1  "<I_pack_A>"
  Truth_sel/6 -> lt_dbl7/1  "<E_out_Wh>"
  Truth_sel/7 -> lt_dbl8/1  "<E_in_Wh>"
  Truth_sel/8 -> lt_dbl9/1  "<E_chg_bus_Wh>"
  Truth_sel/9 -> lt_dbl10/1  "<E_trac_dc_Wh>"
  Truth_sel/10 -> lt_dbl11/1  "<E_impl_dc_Wh>"
  Truth_sel/11 -> lt_dbl12/1  "<E_lv_Wh>"
  Truth_sel/12 -> lt_dbl13/1  "<E_dcdc_loss_Wh>"
  Truth_sel/13 -> lt_dbl14/1  "<E_pdu_loss_Wh>"
  Truth_sel/14 -> lt_dbl15/1  "<E_loss_batt_Wh>"
  Truth_sel/15 -> lt_dbl16/1  "<I_pack_peak_A>"
  Truth_sel/16 -> lt_dbl17/1  "<P_grid_W>"
  SOC_true_min/1 -> lt_dbl18/1  "SOC_true_min"
  V_cell_true_max/1 -> lt_dbl19/1  "V_cell_true_max"
  Clock_100ms_log/1 -> lt_dbl1/1  "t_100ms_log"
  Mcu_log_BC/1 -> Ispd_log_sel/1, Ien_log_sel/1, Hv_log_sel/1  "mcu_log"
  V_drv_R/1 -> V_drv_R_d/1  "V_drv_R"
  V_drv_L/1 -> V_drv_L_d/1  "V_drv_L"
  lt_dbl1/1 -> log_truth_mux/1  "t_dbl"
  lt_dbl2/1 -> log_truth_mux/2  "SOC_pack_true_dbl"
  lt_dbl3/1 -> log_truth_mux/3  "T_cell_max_K_dbl"
  lt_dbl4/1 -> log_truth_mux/4  "T_cell_min_K_dbl"
  lt_dbl5/1 -> log_truth_mux/5  "V_term_V_dbl"
  lt_dbl6/1 -> log_truth_mux/6  "I_pack_A_dbl"
  lt_dbl7/1 -> log_truth_mux/7  "E_out_Wh_dbl"
  lt_dbl8/1 -> log_truth_mux/8  "E_in_Wh_dbl"
  lt_dbl9/1 -> log_truth_mux/9  "E_chg_bus_Wh_dbl"
  lt_dbl10/1 -> log_truth_mux/10  "E_trac_dc_Wh_dbl"
  lt_dbl11/1 -> log_truth_mux/11  "E_impl_dc_Wh_dbl"
  lt_dbl12/1 -> log_truth_mux/12  "E_lv_Wh_dbl"
  lt_dbl13/1 -> log_truth_mux/13  "E_dcdc_loss_Wh_dbl"
  lt_dbl14/1 -> log_truth_mux/14  "E_pdu_loss_Wh_dbl"
  lt_dbl15/1 -> log_truth_mux/15  "E_loss_batt_Wh_dbl"
  lt_dbl16/1 -> log_truth_mux/16  "I_pack_peak_A_dbl"
  lt_dbl17/1 -> log_truth_mux/17  "P_grid_W_dbl"
  lt_dbl18/1 -> log_truth_mux/18  "SOC_true_min_dbl"
  lt_dbl19/1 -> log_truth_mux/19  "V_cell_true_max_dbl"
  BMS/1 -> Power_Plant/4, Cmd_sel/1  "bms_cmd"
  BMS/2 -> can_tx_bms_term/1  "can_tx_bms"
  BMS/3 -> Tel_sel/1  "telem"
  Hv_log_sel/1 -> Hv_RT/1  "<HV_Enable_Req>"
  Ien_log_sel/1 -> Ien_RT/1  "<impl_enable>"
  Ispd_log_sel/1 -> Ispd_RT/1  "<impl_speed_rpm>"
  Tel_sel/1 -> lb_dbl2/1  "<Contactor_State>"
  Tel_sel/2 -> lb_dbl3/1  "<HV_Ready>"
  Tel_sel/3 -> lb_dbl4/1  "<Fault_Level>"
  Tel_sel/4 -> lb_dbl5/1  "<Fault_Word>"
  Tel_sel/5 -> lb_dbl6/1  "<Warning_Word>"
  Tel_sel/6 -> lb_dbl7/1  "<SOC_pack>"
  Tel_sel/7 -> lb_dbl8/1  "<Charging_Active>"
  Tel_sel/8 -> lb_dbl9/1  "<Charge_Complete>"
  Tel_sel/9 -> lb_dbl10/1  "<I_chg_lim_A>"
  Tel_sel/10 -> lb_dbl11/1  "<I_dis_lim_A>"
  Tel_sel/11 -> lb_dbl12/1  "<T_cell_max_K>"
  Tel_sel/12 -> lb_dbl13/1  "<Fan_Cmd>"
  Tel_sel/13 -> lb_dbl14/1  "<K1_Closed>"
  Tel_sel/14 -> lb_dbl15/1  "<Runtime_Remaining_s>"
  Impl_sel/1 -> ls_dbl2/1  "<Impl_Running>"
  Impl_sel/2 -> ls_dbl3/1  "<Impl_Fault>"
  Impl_sel/3 -> ls_dbl4/1  "<Impl_Ready>"
  Impl_sel/4 -> ls_dbl5/1  "<Impl_Speed_radps>"
  Impl_sel/5 -> ls_dbl6/1  "<Impl_Torque_Nm>"
  Impl_sel/6 -> ls_dbl7/1  "<Impl_Power_W>"
  Impl_sel/7 -> ls_dbl8/1  "<Impl_Current_A>"
  Impl_sel/8 -> ls_dbl9/1  "<Fault_Code>"
  Cmd_sel/1 -> ls_dbl10/1  "<K1_Cmd>"
  Cmd_sel/2 -> ls_dbl11/1  "<K2_Cmd>"
  Cmd_sel/3 -> ls_dbl12/1  "<K4_Cmd>"
  Cmd_sel/4 -> ls_dbl13/1  "<Charger_Enable>"
  Cmd_sel/5 -> ls_dbl14/1  "<Charger_I_Req_A>"
  Cmd_sel/6 -> ls_dbl15/1  "<Fan_Cmd>"
  log_truth_mux/1 -> log_truth/1  "log_truth"
  W_impl/1 -> W_impl_d/1  "w_impl"
  V_drv_L_d/1 -> Stub_log_BC/5, V_L_min/1, Gate_L_off/1  "V_drv_L_d"
  Hv_RT/1 -> ls_dbl16/1  "Hv_RT"
  Ien_RT/1 -> ls_dbl17/1  "Ien_RT"
  Ispd_RT/1 -> ls_dbl18/1  "Ispd_RT"
  V_drv_R_d/1 -> Stub_log_BC/6, V_R_min/1, Gate_R_off/1  "V_drv_R_d"
  Clock_100ms_log_bms/1 -> lb_dbl1/1  "t_100ms_log_bms"
  Clock_10ms/1 -> ls_dbl1/1  "t_10ms"
  Clock_base_stub/1 -> LF/1, Load_R/1, Load_L/1, Short/1  "t_base_stub"
  V_R_min/1 -> I_from_P_R/2  "V_drv_R_min"
  V_L_min/1 -> I_from_P_L/2  "V_drv_L_min"
  W_impl_d/1 -> Stub_log_BC/3, W_sq/1, K_lin/1, W_impl_RT/1, W_abs/1, K_lf/1, W_10/1  "w_impl_d"
  Gate_R_off/1 -> Gate_R_k/1  "gate_dV_R"
  Gate_L_off/1 -> Gate_L_k/1  "gate_dV_L"
  Load_R/1 -> Load_mode_R/3, I_from_P_R/1  "load_R"
  Load_L/1 -> Load_mode_L/3, I_from_P_L/1  "load_L"
  lb_dbl1/1 -> log_bms_mux/1  "t_dbl"
  lb_dbl2/1 -> log_bms_mux/2  "Contactor_State_dbl"
  lb_dbl3/1 -> log_bms_mux/3  "HV_Ready_dbl"
  lb_dbl4/1 -> log_bms_mux/4  "Fault_Level_dbl"
  lb_dbl5/1 -> log_bms_mux/5  "Fault_Word_dbl"
  lb_dbl6/1 -> log_bms_mux/6  "Warning_Word_dbl"
  lb_dbl7/1 -> log_bms_mux/7  "SOC_pack_dbl"
  lb_dbl8/1 -> log_bms_mux/8  "Charging_Active_dbl"
  lb_dbl9/1 -> log_bms_mux/9  "Charge_Complete_dbl"
  lb_dbl10/1 -> log_bms_mux/10  "I_chg_lim_A_dbl"
  lb_dbl11/1 -> log_bms_mux/11  "I_dis_lim_A_dbl"
  lb_dbl12/1 -> log_bms_mux/12  "T_cell_max_K_dbl"
  lb_dbl13/1 -> log_bms_mux/13  "Fan_Cmd_dbl"
  lb_dbl14/1 -> log_bms_mux/14  "K1_Closed_dbl"
  lb_dbl15/1 -> log_bms_mux/15  "Runtime_Remaining_s_dbl"
  ls_dbl1/1 -> log_slow_mux/1  "t_dbl"
  ls_dbl2/1 -> log_slow_mux/2  "Impl_Running_dbl"
  ls_dbl3/1 -> log_slow_mux/3  "Impl_Fault_dbl"
  ls_dbl4/1 -> log_slow_mux/4  "Impl_Ready_dbl"
  ls_dbl5/1 -> log_slow_mux/5  "Impl_Speed_radps_dbl"
  ls_dbl6/1 -> log_slow_mux/6  "Impl_Torque_Nm_dbl"
  ls_dbl7/1 -> log_slow_mux/7  "Impl_Power_W_dbl"
  ls_dbl8/1 -> log_slow_mux/8  "Impl_Current_A_dbl"
  ls_dbl9/1 -> log_slow_mux/9  "Fault_Code_dbl"
  ls_dbl10/1 -> log_slow_mux/10  "K1_Cmd_dbl"
  ls_dbl11/1 -> log_slow_mux/11  "K2_Cmd_dbl"
  ls_dbl12/1 -> log_slow_mux/12  "K4_Cmd_dbl"
  ls_dbl13/1 -> log_slow_mux/13  "Charger_Enable_dbl"
  ls_dbl14/1 -> log_slow_mux/14  "Charger_I_Req_A_dbl"
  ls_dbl15/1 -> log_slow_mux/15  "Fan_Cmd_dbl"
  ls_dbl16/1 -> log_slow_mux/16  "HV_Enable_Req_10ms_dbl"
  ls_dbl17/1 -> log_slow_mux/17  "impl_enable_10ms_dbl"
  ls_dbl18/1 -> log_slow_mux/18  "impl_speed_rpm_10ms_dbl"
  log_bms_mux/1 -> log_bms/1  "log_bms"
  log_slow_mux/1 -> log_slow/1  "log_slow"
  I_from_P_R/1 -> Load_mode_R/1  "I_from_P_R"
  Is_power_R/1 -> Load_mode_R/2  "load_is_power_R"
  Gate_R_k/1 -> Gate_R/1  "gate_raw_R"
  I_from_P_L/1 -> Load_mode_L/1  "I_from_P_L"
  Is_power_L/1 -> Load_mode_L/2  "load_is_power_L"
  Gate_L_k/1 -> Gate_L/1  "gate_raw_L"
  W_10/1 -> W_sat/1  "w_impl_10"
  Short/1 -> Short_PS/1  "short_cmd"
  Gate_R/1 -> I_load_R/2  "gate_R"
  Gate_L/1 -> I_load_L/2  "gate_L"
  W_sat/1 -> T_c/1  "w_impl_sign"
  Load_mode_R/1 -> I_load_R/1  "I_load_req_R"
  Load_mode_L/1 -> I_load_L/1  "I_load_req_L"
  W_abs/1 -> W_sq/2  "w_impl_abs"
  I_load_L/1 -> Stub_log_BC/1, I_drv_L_PS/1  "I_load_L"
  T_c/1 -> T_lf_sum/1  "T_coulomb"
  K_lf/1 -> T_lf_sum/2  "T_lf_lin"
  I_load_R/1 -> Stub_log_BC/2, I_drv_R_PS/1  "I_load_R"
  T_lf_sum/1 -> T_lf/1  "T_lf_base"
  W_sq/1 -> K_aero/1  "w_impl_sq"
  LF/1 -> T_lf/2  "load_factor"
  K_aero/1 -> T_load/1  "T_aero"
  K_lin/1 -> T_load/2  "T_lin"
  T_lf/1 -> T_load/3  "T_lf"
  W_impl_RT/1 -> Mech_BA/3, W_sq_p/2, W_sq_p/1  "w_impl_10ms"
  T_load/1 -> Stub_log_BC/4, T_load_PS/1, T_load_RT/1  "T_load"
  W_sq_p/1 -> P_line/1  "w_impl_sq_10ms"
  Stub_log_BC/1 -> Stub_log_sel/1  "stub_log"
  Mech_ic/1 -> Mech_BA/1  "impl_mech_ic"
  Impl_type/1 -> Mech_BA/2  "impl_type"
  P_line/1 -> Mech_BA/5  "line_pressure"
  T_load_RT/1 -> Mech_BA/4  "T_load_10ms"
  Status_sel/1 -> lf_dbl2/1  "<V_pack_V>"
  Status_sel/2 -> lf_dbl3/1  "<I_pack_A>"
  Status_sel/3 -> lf_dbl4/1  "<V_bus_V>"
  Status_sel/4 -> lf_dbl5/1  "<V_24V_V>"
  Status_sel/5 -> lf_dbl6/1  "<I_24V_A>"
  Status_sel/6 -> lf_dbl7/1  "<V_24IMP_V>"
  Status_sel/7 -> lf_dbl8/1  "<V_12V_V>"
  Status_sel/8 -> lf_dbl9/1  "<I_12V_A>"
  Status_sel/9 -> lf_dbl10/1  "<V_5V_V>"
  Status_sel/10 -> lf_dbl11/1  "<V_3V3_V>"
  Status_sel/11 -> lf_dbl12/1  "<Rail_24V_OK>"
  Status_sel/12 -> lf_dbl13/1  "<Rail_12V_OK>"
  Status_sel/13 -> lf_dbl14/1  "<Rail_5V_OK>"
  Status_sel/14 -> lf_dbl15/1  "<Rail_3V3_OK>"
  Status_sel/15 -> lf_dbl16/1  "<K1_Closed>"
  Status_sel/16 -> lf_dbl17/1  "<K2_Closed>"
  Status_sel/17 -> lf_dbl18/1  "<K3_Closed>"
  Status_sel/18 -> lf_dbl19/1  "<K4_Closed>"
  Status_sel/19 -> lf_dbl20/1  "<Safety_OK>"
  Status_sel/20 -> lf_dbl21/1  "<Safety_HV_OK>"
  Status_sel/21 -> lf_dbl22/1  "<EStop_Any>"
  Status_sel/22 -> lf_dbl23/1  "<EStop_Ch1_OK>"
  Status_sel/23 -> lf_dbl24/1  "<EStop_Ch2_OK>"
  Status_sel/24 -> lf_dbl25/1  "<Safety_Latched_Off>"
  Status_sel/25 -> lf_dbl26/1  "<Dock_Present>"
  Status_sel/26 -> lf_dbl27/1  "<Key_On>"
  Status_sel/27 -> lf_dbl28/1  "<Fuse_Blown>"
  Stub_log_sel/1 -> lf_dbl29/1  "<I_load_L>"
  Stub_log_sel/2 -> lf_dbl30/1  "<I_load_R>"
  Stub_log_sel/3 -> lf_dbl31/1  "<w_impl_d>"
  Stub_log_sel/4 -> lf_dbl32/1  "<T_load>"
  Stub_log_sel/5 -> lf_dbl33/1  "<V_drv_L_d>"
  Stub_log_sel/6 -> lf_dbl34/1  "<V_drv_R_d>"
  Mech_BA/1 -> Power_Plant/6  "impl_mech"
  Clock_base/1 -> lf_dbl1/1  "t_base"
  lf_dbl1/1 -> log_fast_mux/1  "t_dbl"
  lf_dbl2/1 -> log_fast_mux/2  "V_pack_V_dbl"
  lf_dbl3/1 -> log_fast_mux/3  "I_pack_A_dbl"
  lf_dbl4/1 -> log_fast_mux/4  "V_bus_V_dbl"
  lf_dbl5/1 -> log_fast_mux/5  "V_24V_V_dbl"
  lf_dbl6/1 -> log_fast_mux/6  "I_24V_A_dbl"
  lf_dbl7/1 -> log_fast_mux/7  "V_24IMP_V_dbl"
  lf_dbl8/1 -> log_fast_mux/8  "V_12V_V_dbl"
  lf_dbl9/1 -> log_fast_mux/9  "I_12V_A_dbl"
  lf_dbl10/1 -> log_fast_mux/10  "V_5V_V_dbl"
  lf_dbl11/1 -> log_fast_mux/11  "V_3V3_V_dbl"
  lf_dbl12/1 -> log_fast_mux/12  "Rail_24V_OK_dbl"
  lf_dbl13/1 -> log_fast_mux/13  "Rail_12V_OK_dbl"
  lf_dbl14/1 -> log_fast_mux/14  "Rail_5V_OK_dbl"
  lf_dbl15/1 -> log_fast_mux/15  "Rail_3V3_OK_dbl"
  lf_dbl16/1 -> log_fast_mux/16  "K1_Closed_dbl"
  lf_dbl17/1 -> log_fast_mux/17  "K2_Closed_dbl"
  lf_dbl18/1 -> log_fast_mux/18  "K3_Closed_dbl"
  lf_dbl19/1 -> log_fast_mux/19  "K4_Closed_dbl"
  lf_dbl20/1 -> log_fast_mux/20  "Safety_OK_dbl"
  lf_dbl21/1 -> log_fast_mux/21  "Safety_HV_OK_dbl"
  lf_dbl22/1 -> log_fast_mux/22  "EStop_Any_dbl"
  lf_dbl23/1 -> log_fast_mux/23  "EStop_Ch1_OK_dbl"
  lf_dbl24/1 -> log_fast_mux/24  "EStop_Ch2_OK_dbl"
  lf_dbl25/1 -> log_fast_mux/25  "Safety_Latched_Off_dbl"
  lf_dbl26/1 -> log_fast_mux/26  "Dock_Present_dbl"
  lf_dbl27/1 -> log_fast_mux/27  "Key_On_dbl"
  lf_dbl28/1 -> log_fast_mux/28  "Fuse_Blown_dbl"
  lf_dbl29/1 -> log_fast_mux/29  "I_load_L_dbl"
  lf_dbl30/1 -> log_fast_mux/30  "I_load_R_dbl"
  lf_dbl31/1 -> log_fast_mux/31  "w_impl_d_dbl"
  lf_dbl32/1 -> log_fast_mux/32  "T_load_dbl"
  lf_dbl33/1 -> log_fast_mux/33  "V_drv_L_d_dbl"
  lf_dbl34/1 -> log_fast_mux/34  "V_drv_R_d_dbl"
  log_fast_mux/1 -> log_fast/1  "log_fast"
  connections:
  W_impl_sens/RConn3 -- Angle_term/LConn1
  V_drv_L_sens/LConn1 -- Power_Plant/RConn1 -- S_short/LConn2 -- I_drv_L/RConn2 -- C_drv_L/LConn1
  Solver/RConn1 -- Power_Plant/RConn2 -- V_drv_L_sens/RConn2 -- R_short/RConn1 -- I_drv_L/LConn1 -- C_drv_L/RConn1
  V_drv_R_sens/LConn1 -- Power_Plant/RConn3 -- C_drv_R/LConn1 -- I_drv_R/RConn2
  V_drv_R_sens/RConn2 -- Power_Plant/RConn4 -- C_drv_R/RConn1 -- I_drv_R/LConn1
  I_drv_L_PS/RConn1 -- I_drv_L/RConn1
  I_drv_R_PS/RConn1 -- I_drv_R/RConn1
  J_impl/LConn1 -- Power_Plant/RConn5 -- W_impl_sens/LConn1 -- T_load_src/LConn1
  S_short/RConn1 -- R_short/LConn1
  Ref_impl/LConn1 -- W_impl_sens/RConn1 -- T_load_src/RConn2
  Short_PS/RConn1 -- S_short/LConn1
  T_load_PS/RConn1 -- T_load_src/RConn1
  V_drv_L_sens/RConn1 -- V_drv_L/LConn1
  V_drv_R/LConn1 -- V_drv_R_sens/RConn1
  W_impl_sens/RConn2 -- W_impl/LConn1
